simulink model "BLDCSpeedControl_EV_Layout_v2_before_step1"  (R2024b)
settings: Solver=ode23t  StartTime=0.0  StopTime=0.3  FixedStep=Ts  MaxStep=5e-4  RelTol=1e-3  EnableMultiTasking=on
PreLoadFcn:
  | BLDCSpeedControlData;
InitFcn:
  | % [EV_DAQ_V7_HOOK]
  | try; EV_DAQ_Builder_V7('Overrides'); catch ME__daq; fprintf('[DAQ] Overrides error: %s\n', ME__daq.message); end
StartFcn:
  | % [EV_DAQ_V7_HOOK]
  | try; EV_DAQ_Builder_V7('AutoInit'); catch ME__daq; fprintf('[DAQ] Auto-init error: %s\n', ME__daq.message); end
StopFcn:
  | % [EV_DAQ_V7_HOOK]
  | try; EV_DAQ_Builder_V7('PostProcess'); catch ME__daq; fprintf('[DAQ] Post-process error: %s\n', ME__daq.message); end
values from neighbouring files (symbols this model uses):
  Emax = (P.I_peak^2 - P.I_cont^2)*safeBase('t_peak',1)    [EV_DAQ_Builder_V7_BACKUP_20261009_124326.m]    (also in EV_DAQ_Builder_V7_ORIGINAL_BACKUP.m)
  m = get_param(blk,'Multiplication')    [EV_DAQ_Builder_V7_BACKUP_20261009_124326.m]    (also in EV_DAQ_Builder_V7_ORIGINAL_BACKUP.m)
  N = comp.N    [EV_DAQ_Builder_V7_BACKUP_20261009_124326.m]    (also in EV_DAQ_Builder_V7_ORIGINAL_BACKUP.m)
  p = sprintf('    [EV_DAQ_Builder_V7_BACKUP_20261009_124326.m]    (also in EV_DAQ_Builder_V7_ORIGINAL_BACKUP.m)
  s = [char(65 + r) s]    [EV_DAQ_Builder_V7_BACKUP_20261009_124326.m]    (also in EV_DAQ_Builder_V7_ORIGINAL_BACKUP.m)
undefined symbols (not defined in the file or in its folder): battery_builder_rtmsupport, cells_parallel, cells_series, DiscIntNeverNeededParam, Emax_thr, emf_max_ev, gcbh, I_cont, I_peak, Ke_ph, Kii, Kiv, Kiw, Kpi, Kpv, Kpw, load_scale, r_wheel, rpm_ramp, rpm_ref, T_Ifilt, Ts, Tsc, Vdc, Vlim_min, wheel_mass
libraries: nesl_utility x19, fl_lib x13, ee_lib x6, sm_lib x3, eeDiscretePi x2, Batteries2_lib x1, SignalEditorBlockLib x1, eePwmGenerator x1, eeGeneralControl x1
(part 2 of 2)

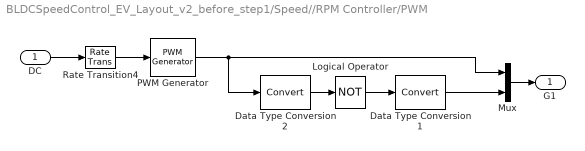
== system BLDCSpeedControl_EV_Layout_v2_before_step1/Speed//RPM Controller/PWM ==
  DC : Inport
  Data Type Conversion1 : DataTypeConversion  SaturateOnIntegerOverflow=off  RndMeth=Floor
  Data Type Conversion2 : DataTypeConversion  SaturateOnIntegerOverflow=off  RndMeth=Floor
  Logical Operator : Logic  Operator=NOT  AllPortsSameDT=off  OutDataTypeStr=boolean
  Mux : Mux  Inputs=2
  PWM Generator : eePwmGenerator/PWM Generator  CarrCount=Up  Tper=Tsc  Tdelay=0  Ts=Ts
  Rate Transition4 : RateTransition  OutPortSampleTime=Ts
  G1 : Outport  VectorParamsAs1DForOutWhenUnconnected=off
  wires:
  Mux/1 -> G1/1
  Rate Transition4/1 -> PWM Generator/1
  PWM Generator/1 -> Data Type Conversion2/1, Mux/1
  Data Type Conversion1/1 -> Mux/2
  Logical Operator/1 -> Data Type Conversion1/1
  DC/1 -> Rate Transition4/1
  Data Type Conversion2/1 -> Logical Operator/1

== system BLDCSpeedControl_EV_Layout_v2_before_step1/Speed//RPM Controller/Sign ==
  u : Inport
  Constant2 : Constant
  Constant3 : Constant  Value=-1
  Switch : Switch  SaturateOnIntegerOverflow=off  InputSameDT=off
  y : Outport
  wires:
  Constant3/1 -> Switch/3
  Constant2/1 -> Switch/1
  u/1 -> Switch/2
  Switch/1 -> y/1

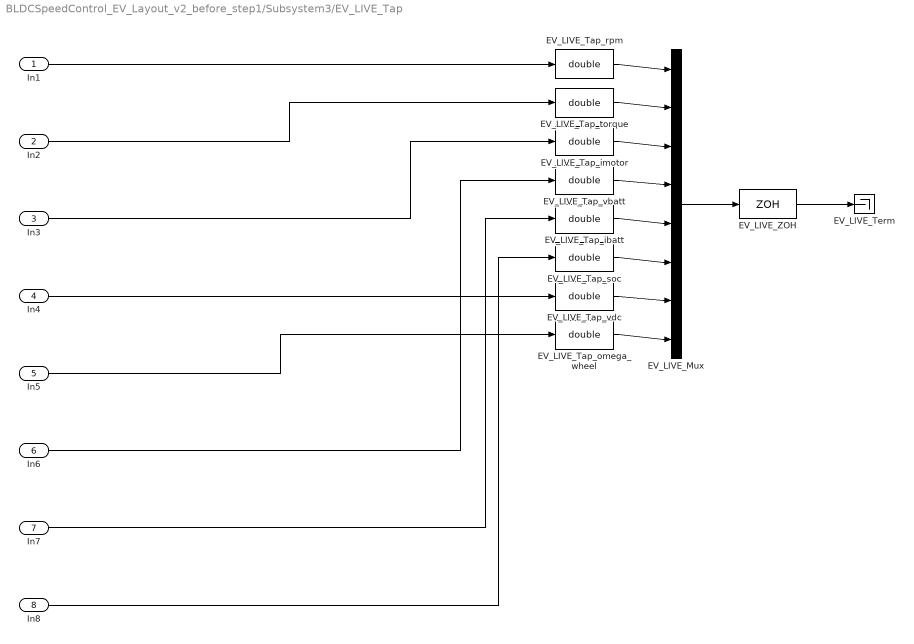
== system BLDCSpeedControl_EV_Layout_v2_before_step1/Subsystem3/EV_LIVE_Tap ==
  In1 : Inport
  In2 : Inport  Port=2
  In3 : Inport  Port=3
  In4 : Inport  Port=4
  In5 : Inport  Port=5
  In6 : Inport  Port=6
  In7 : Inport  Port=7
  In8 : Inport  Port=8
  EV_LIVE_Mux : Mux  Inputs=8
  EV_LIVE_Tap_ibatt : DataTypeConversion  OutDataTypeStr=double
  EV_LIVE_Tap_imotor : DataTypeConversion  OutDataTypeStr=double
  EV_LIVE_Tap_omega_wheel : DataTypeConversion  OutDataTypeStr=double
  EV_LIVE_Tap_rpm : DataTypeConversion  OutDataTypeStr=double
  EV_LIVE_Tap_soc : DataTypeConversion  OutDataTypeStr=double
  EV_LIVE_Tap_torque : DataTypeConversion  OutDataTypeStr=double
  EV_LIVE_Tap_vbatt : DataTypeConversion  OutDataTypeStr=double
  EV_LIVE_Tap_vdc : DataTypeConversion  OutDataTypeStr=double
  EV_LIVE_Term : Terminator
  EV_LIVE_ZOH : ZeroOrderHold  SampleTime=0.1
  wires:
  EV_LIVE_Mux/1 -> EV_LIVE_ZOH/1
  EV_LIVE_Tap_rpm/1 -> EV_LIVE_Mux/1
  In5/1 -> EV_LIVE_Tap_omega_wheel/1
  EV_LIVE_Tap_imotor/1 -> EV_LIVE_Mux/3
  EV_LIVE_ZOH/1 -> EV_LIVE_Term/1
  EV_LIVE_Tap_torque/1 -> EV_LIVE_Mux/2
  EV_LIVE_Tap_ibatt/1 -> EV_LIVE_Mux/5
  In6/1 -> EV_LIVE_Tap_vbatt/1
  EV_LIVE_Tap_vbatt/1 -> EV_LIVE_Mux/4
  EV_LIVE_Tap_omega_wheel/1 -> EV_LIVE_Mux/8
  EV_LIVE_Tap_soc/1 -> EV_LIVE_Mux/6
  EV_LIVE_Tap_vdc/1 -> EV_LIVE_Mux/7
  In8/1 -> EV_LIVE_Tap_soc/1
  In1/1 -> EV_LIVE_Tap_rpm/1
  In2/1 -> EV_LIVE_Tap_torque/1
  In4/1 -> EV_LIVE_Tap_vdc/1
  In3/1 -> EV_LIVE_Tap_imotor/1
  In7/1 -> EV_LIVE_Tap_ibatt/1

== system BLDCSpeedControl_EV_Layout_v2_before_step1/Subsystem3/Subsystem ==
  In1 : Inport
  In2 : Inport  Port=2
  In3 : Inport  Port=3
  In4 : Inport  Port=4
  In5 : Inport  Port=5
  In6 : Inport  Port=6
  In7 : Inport  Port=7

== system BLDCSpeedControl_EV_Layout_v2_before_step1/Subsystem3/Subsystem1 ==
  In1 : Inport
  In2 : Inport  Port=2
  In3 : Inport  Port=3
  In4 : Inport  Port=4
  In5 : Inport  Port=5
  In6 : Inport  Port=6
  In7 : Inport  Port=7
  In8 : Inport  Port=8

== system BLDCSpeedControl_EV_Layout_v2_before_step1/Subsystem3/Subsystem2 ==
  In1 : Inport
  In2 : Inport  Port=2
  In3 : Inport  Port=3
  In4 : Inport  Port=4
  In5 : Inport  Port=5
  In6 : Inport  Port=6
  In7 : Inport  Port=7
  In8 : Inport  Port=8

== system BLDCSpeedControl_EV_Layout_v2_before_step1/Sensing w a/Hall sensor/Subsystem ==
  theta : Inport
  Trigonometric Function : Trigonometry  Operator=sincos
  Trigonometric Function2 : Trigonometry  Operator=atan2
  mech->elec : Gain  Gain=p
  rad->deg : Gain  Gain=180/pi  SaturateOnIntegerOverflow=on  OutDataTypeStr=Inherit: Same as input  ParamDataTypeStr=Inherit: Same as input
  deg : Outport  VectorParamsAs1DForOutWhenUnconnected=off
  wires:
  Trigonometric Function2/1 -> rad->deg/1
  Trigonometric Function/1 -> Trigonometric Function2/1
  theta/1 -> mech->elec/1
  rad->deg/1 -> deg/1
  Trigonometric Function/2 -> Trigonometric Function2/2
  mech->elec/1 -> Trigonometric Function/1

== system BLDCSpeedControl_EV_Layout_v2_before_step1/Speed//RPM Controller/Commutation/Bit concatenate ==
  u : Inport
  Gain : Gain  Gain=[4 2 1]  Multiplication=Matrix(K*u)
  Sum of Elements : Sum  Inputs=+
  y : Outport  VectorParamsAs1DForOutWhenUnconnected=off
  wires:
  u/1 -> Gain/1
  Gain/1 -> Sum of Elements/1
  Sum of Elements/1 -> y/1
